simulink model "profacccomplex_sim"  (R2026a)
settings: Solver=ode45  StopTime=180
settings Model: Creator=sprinkle  LastModifiedBy=sprinkle

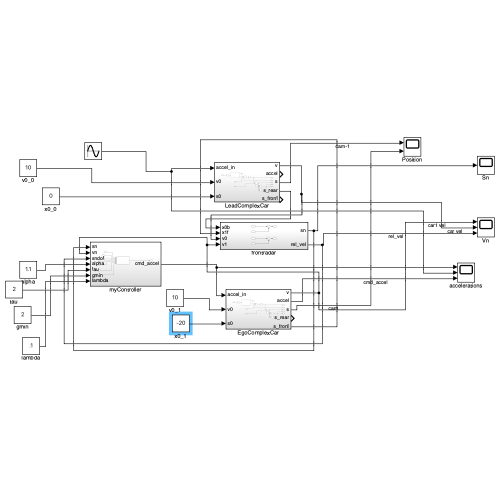
[thumbnail: Simulink's stored preview of the top-level diagram]
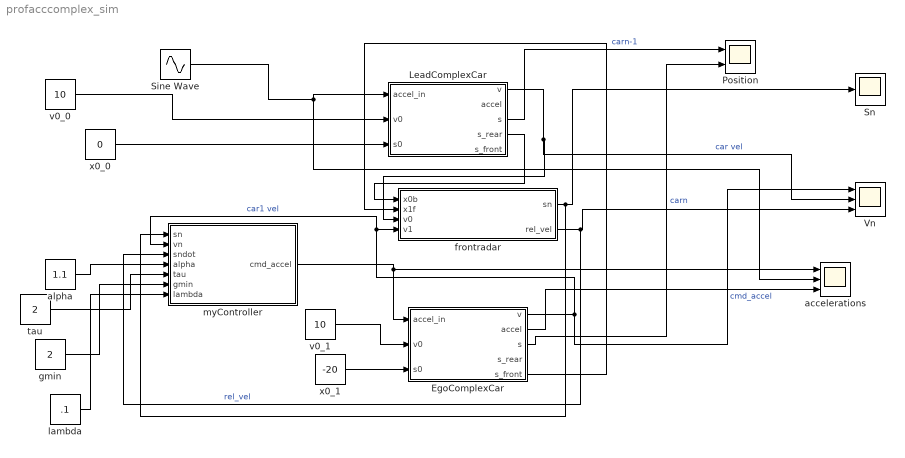
== system profacccomplex_sim ==
  EgoComplexCar : Subsystem
  LeadComplexCar : Subsystem
  Position : Scope  NumInputPorts=2
      settings: ActiveDisplayYMinimum=-44.355853288409918  ActiveDisplayYMaximum=452.73687301845121  DataLoggingVariableName=ScopeData3
  Sine Wave : Sin  Amplitude=0.5  SampleTime=0
  Sn : Scope
      settings: ActiveDisplayYMinimum=-16.103354872680892  ActiveDisplayYMaximum=84.114102258000287
  Vn : Scope  NumInputPorts=3
      settings: ActiveDisplayYMinimum=-15.138495740337117  ActiveDisplayYMaximum=35.655531147670587
  accelerations : Scope  NumInputPorts=3
      settings: ActiveDisplayYMinimum=-2.940561369613075  ActiveDisplayYMaximum=1.1550844027430727  DataLoggingVariableName=ScopeData2
  alpha : Constant  Value=1.1
  frontradar : Subsystem
  gmin : Constant  Value=2
  lambda : Constant  Value=.1
  myController : Subsystem
  tau : Constant  Value=2
  v0_0 : Constant  Value=10
  v0_1 : Constant  Value=10
  x0_0 : Constant  Value=0
  x0_1 : Constant  Value=-20
  wires:
  Sine Wave/1 -> LeadComplexCar/1(accel_in), accelerations/2
  v0_0/1 -> LeadComplexCar/2(v0)
  x0_0/1 -> LeadComplexCar/3(s0)
  LeadComplexCar/4(s_rear) -> frontradar/1(x0b)
  EgoComplexCar/5(s_front) -> frontradar/2(x1f)
  LeadComplexCar/1(v) -> Vn/2, frontradar/3(v0)  "car vel"
  EgoComplexCar/1(v) -> Vn/1, myController/2(vn), frontradar/4(v1)  "car1 vel"
  frontradar/1(sn) -> myController/1(sn), Sn/1
  frontradar/2(rel_vel) -> myController/3(sndot), Vn/3  "rel_vel"
  alpha/1 -> myController/4(alpha)
  tau/1 -> myController/5(tau)
  myController/1(cmd_accel) -> EgoComplexCar/1(accel_in), accelerations/1
  v0_1/1 -> EgoComplexCar/2(v0)
  x0_1/1 -> EgoComplexCar/3(s0)
  EgoComplexCar/2(accel) -> accelerations/3  "cmd_accel"
  gmin/1 -> myController/6(gmin)
  lambda/1 -> myController/7(lambda)
  LeadComplexCar/3(s) -> Position/1  "carn-1"
  EgoComplexCar/3(s) -> Position/2  "carn"

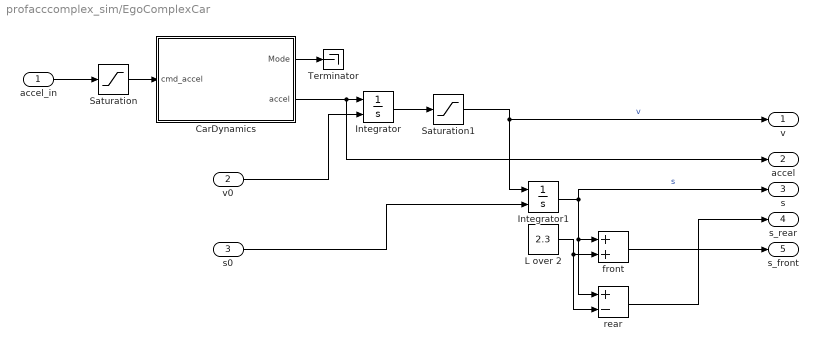
== system profacccomplex_sim/EgoComplexCar ==
  accel_in : Inport
  v0 : Inport  Port=2
  s0 : Inport  Port=3
  CarDynamics : Subsystem
  Integrator : Integrator  InitialConditionSource=external
  Integrator1 : Integrator  InitialConditionSource=external
  L over 2 : Constant  Value=2.3
  Saturation : Saturate  UpperLimit=1.5  LowerLimit=-3.5
  Saturation1 : Saturate  UpperLimit=30  LowerLimit=0
  Terminator : Terminator
  front : Sum
  rear : Sum  Inputs=+-
  v : Outport
  accel : Outport  Port=2
  s : Outport  Port=3
  s_rear : Outport  Port=4
  s_front : Outport  Port=5
  wires:
  front/1 -> s_front/1
  s0/1 -> Integrator1/2
  CarDynamics/2(accel) -> accel/1, Integrator/1
  v0/1 -> Integrator/2
  L over 2/1 -> rear/2, front/2
  Saturation1/1 -> Integrator1/1, v/1  "v"
  rear/1 -> s_rear/1
  Integrator/1 -> Saturation1/1
  Integrator1/1 -> s/1, rear/1, front/1  "s"
  CarDynamics/1(Mode) -> Terminator/1
  accel_in/1 -> Saturation/1
  Saturation/1 -> CarDynamics/1(cmd_accel)

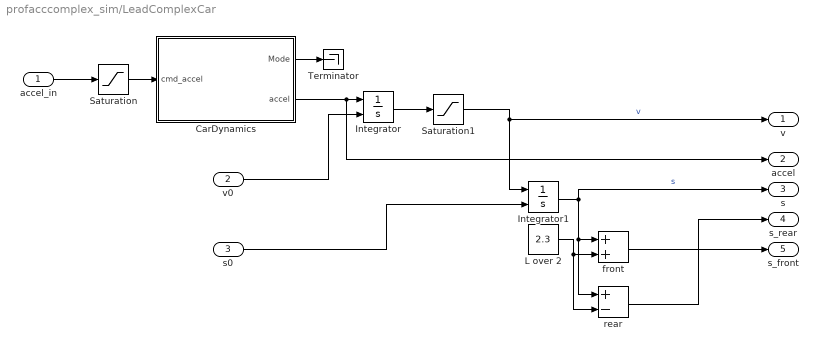
== system profacccomplex_sim/LeadComplexCar ==
  accel_in : Inport
  v0 : Inport  Port=2
  s0 : Inport  Port=3
  CarDynamics : Subsystem
  Integrator : Integrator  InitialConditionSource=external
  Integrator1 : Integrator  InitialConditionSource=external
  L over 2 : Constant  Value=2.3
  Saturation : Saturate  UpperLimit=1.5  LowerLimit=-3.5
  Saturation1 : Saturate  UpperLimit=30  LowerLimit=0
  Terminator : Terminator
  front : Sum
  rear : Sum  Inputs=+-
  v : Outport
  accel : Outport  Port=2
  s : Outport  Port=3
  s_rear : Outport  Port=4
  s_front : Outport  Port=5
  wires:
  front/1 -> s_front/1
  s0/1 -> Integrator1/2
  CarDynamics/2(accel) -> accel/1, Integrator/1
  v0/1 -> Integrator/2
  L over 2/1 -> rear/2, front/2
  Saturation1/1 -> Integrator1/1, v/1  "v"
  rear/1 -> s_rear/1
  Integrator/1 -> Saturation1/1
  Integrator1/1 -> s/1, rear/1, front/1  "s"
  CarDynamics/1(Mode) -> Terminator/1
  accel_in/1 -> Saturation/1
  Saturation/1 -> CarDynamics/1(cmd_accel)

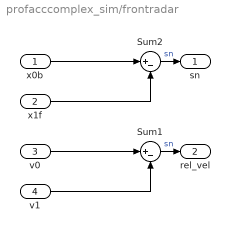
== system profacccomplex_sim/frontradar ==
  x0b : Inport
  x1f : Inport  Port=2
  v0 : Inport  Port=3
  v1 : Inport  Port=4
  Sum1 : Sum  Inputs=|+-
  Sum2 : Sum  Inputs=|+-
  sn : Outport
  rel_vel : Outport  Port=2
  wires:
  x1f/1 -> Sum2/2
  Sum2/1 -> sn/1  "sn"
  x0b/1 -> Sum2/1
  v0/1 -> Sum1/1
  Sum1/1 -> rel_vel/1  "sn"
  v1/1 -> Sum1/2

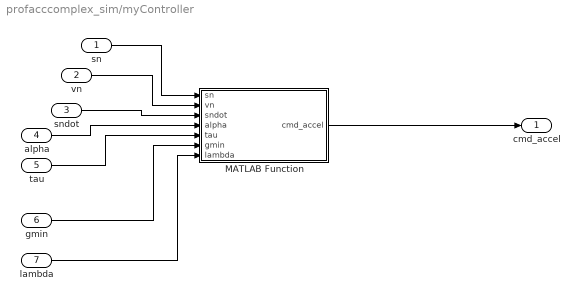
== system profacccomplex_sim/myController ==
  sn : Inport
  vn : Inport  Port=2
  sndot : Inport  Port=3
  alpha : Inport  Port=4
  tau : Inport  Port=5
  gmin : Inport  Port=6
  lambda : Inport  Port=7
  MATLAB Function : MATLAB Function  TreatAsAtomicUnit=on
  cmd_accel : Outport
  wires:
  MATLAB Function/1(cmd_accel) -> cmd_accel/1
  tau/1 -> MATLAB Function/5(tau)
  alpha/1 -> MATLAB Function/4(alpha)
  sn/1 -> MATLAB Function/1(sn)
  vn/1 -> MATLAB Function/2(vn)
  sndot/1 -> MATLAB Function/3(sndot)
  gmin/1 -> MATLAB Function/6(gmin)
  lambda/1 -> MATLAB Function/7(lambda)

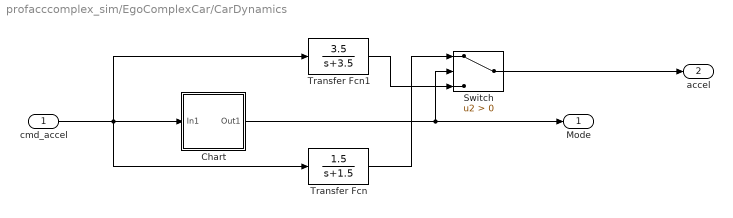
== system profacccomplex_sim/EgoComplexCar/CarDynamics ==
  cmd_accel : Inport
  Chart : Stateflow chart  TreatAsAtomicUnit=on
  Switch : Switch  Criteria=u2 > Threshold  SaturateOnIntegerOverflow=off  InputSameDT=off
  Transfer Fcn : TransferFcn  Numerator=[1.5]  Denominator=[1 1.5]
  Transfer Fcn1 : TransferFcn  Numerator=[3.5]  Denominator=[1 3.5]
  Mode : Outport
  accel : Outport  Port=2
  wires:
  cmd_accel/1 -> Chart/1(In1), Transfer Fcn/1, Transfer Fcn1/1
  Transfer Fcn1/1 -> Switch/3
  Switch/1 -> accel/1
  Transfer Fcn/1 -> Switch/1
  Chart/1(Out1) -> Mode/1, Switch/2

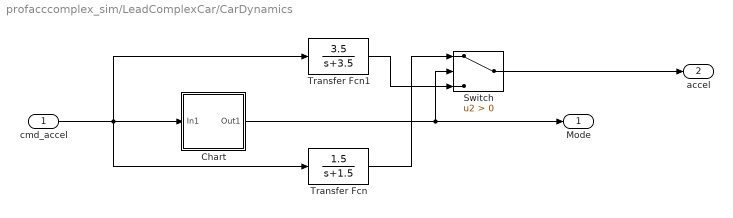
== system profacccomplex_sim/LeadComplexCar/CarDynamics ==
  cmd_accel : Inport
  Chart : Stateflow chart  TreatAsAtomicUnit=on
  Switch : Switch  Criteria=u2 > Threshold  SaturateOnIntegerOverflow=off  InputSameDT=off
  Transfer Fcn : TransferFcn  Numerator=[1.5]  Denominator=[1 1.5]
  Transfer Fcn1 : TransferFcn  Numerator=[3.5]  Denominator=[1 3.5]
  Mode : Outport
  accel : Outport  Port=2
  wires:
  cmd_accel/1 -> Chart/1(In1), Transfer Fcn/1, Transfer Fcn1/1
  Transfer Fcn1/1 -> Switch/3
  Switch/1 -> accel/1
  Transfer Fcn/1 -> Switch/1
  Chart/1(Out1) -> Mode/1, Switch/2

== stateflow chart profacccomplex_sim/EgoComplexCar/CarDynamics/Chart ==
  state Default
    entry: Out1=1;
  state Slowing
    entry: Out1=-1;
  (default) -> Default
  Slowing -> Default : [In1 > 0]
  Default -> Slowing : [In1 < 0.2]
  data: In1 input; Out1 output

== matlab function profacccomplex_sim/myController/MATLAB Function ==
  data: sn input; cmd_accel output; vn input; sndot input; alpha input; tau input; gmin input; lambda input
function cmd_accel = fcn(sn,vn,sndot,alpha,tau,gmin,lambda)
                    
cmd_accel = alpha * (sn - tau*vn - gmin) + lambda*sndot;

== stateflow chart profacccomplex_sim/LeadComplexCar/CarDynamics/Chart ==
  state Default
    entry: Out1=1;
  state Slowing
    entry: Out1=-1;
  (default) -> Default
  Slowing -> Default : [In1 > 0]
  Default -> Slowing : [In1 < 0.2]
  data: In1 input; Out1 output
